simulink model "furuta_pi_motor_speed_a2"  (R2026b)
settings: Solver=FixedStepDiscrete  StopTime=inf  FixedStep=0.005  EnableMultiTasking=on
model workspace (MAT data in the model file):
  calibration = [nan -1 4058.5 1]
  drive = [0 0 0 0]
  limits = [0 0 15 0]
  motorSpeedRPM = Simulink.Parameter
  motorSpeedRPM.Value = 0
  motorSpeedRPM.Complexity = 'real'
  motorSpeedRPM.Dimensions = [1 1]
  motorSpeedRPM.CoderInfo.StorageClass = 'ExportedGlobal'
  motorSpeedRPM.DataType = 'double'
  speedSettings = [0 inf]
libraries: raspberrypiCommlib x5
settings Model: Creator=Lsh  LastModifiedBy=Lsh
settings SolverCC: PositivePriorityOrder=on
settings OptimizationCC: DifferentSizesBufferReuse=on  EfficientTunableParamExpr=on  EnhancedBackFolding=on  MaxStackSize=200000  OptimizationCustomize=off  OptimizeBlockOrder=speed  PassReuseOutputArgsAs=Individual arguments  RemoveInternalMemoryZeroInit=on  RemoveRootLevelIOMemoryZeroInit=on
settings DebuggingCC: ParameterTunabilityLossMsg=error
settings HardwareCC: ProdHWDeviceType=ARM Compatible->ARM Cortex-A (64-bit)  ProdLargestAtomicFloat=Double  ProdLargestAtomicInteger=LongLong  ProdLongLongMode=on
settings RTWCC: BuildConfiguration=Faster Runs  Description=Embedded Coder  HardwareBoard=Raspberry Pi (64bit)  SystemTargetFile=ert.tlc  TLCOptions="-aInlineSetEventsForThisBaseRateFcn=TLC_FALSE -aSuppressMultiTaskScheduler=TLC_FALSE  -aRateBasedStepFcn=0"  TemplateMakefile=ert_default_tmf  Toolchain=GNU GCC RPIUtils
settings CodeAppCC: ForceParamTrailComments=on  IgnoreCustomStorageClasses=off  InsertBlockDesc=on  OperatorAnnotations=on  SFDataObjDesc=on  SimulinkDataObjDesc=on
settings ERTTargetCC: CombineSignalStateStructs=on  ExtModeIntrfLevel=Level2 - Open  ExtModeMexFile=ext_xcp  ExtModeStaticAlloc=on  SupportVariableSizeSignals=on

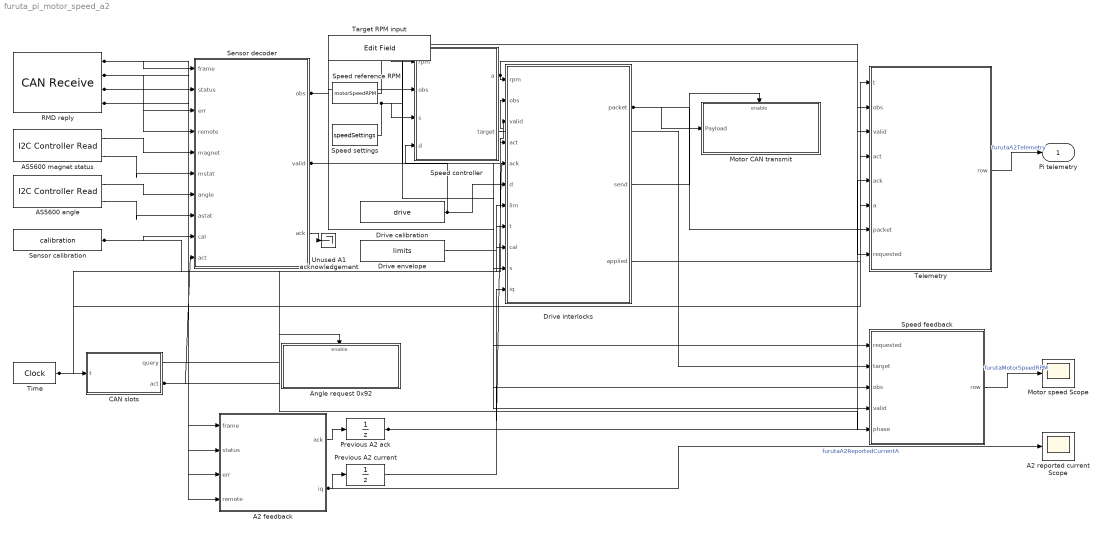
== system furuta_pi_motor_speed_a2 ==
  A2 feedback : MATLAB Function  TreatAsAtomicUnit=on
  A2 reported current Scope : Scope
  AS5600 angle : raspberrypiCommlib/I2C Controller Read  BoardProperty=Pi 5 Model  I2CModule=1  Mode=Master  SlaveAddress=54  SlaveByteOrder=BigEndian  Direction=Receiver  RegisterAddressMode=on  RegisterAddress=14  SlaveDataType=uint8  DataLength=2  NoAck=off  RepeatedStart=on  OutputStatus=on  SampleTime=.005
  AS5600 magnet status : raspberrypiCommlib/I2C Controller Read  BoardProperty=Pi 5 Model  I2CModule=1  Mode=Master  SlaveAddress=54  SlaveByteOrder=BigEndian  Direction=Receiver  RegisterAddressMode=on  RegisterAddress=11  SlaveDataType=uint8  DataLength=1  NoAck=off  RepeatedStart=on  OutputStatus=on  SampleTime=.005
  Angle request 0x92 : Subsystem  TreatAsAtomicUnit=on
  CAN slots : MATLAB Function  TreatAsAtomicUnit=on
  Drive calibration : Constant  Value=drive  SampleTime=.005
  Drive envelope : Constant  Value=limits  SampleTime=.005
  Drive interlocks : MATLAB Function  TreatAsAtomicUnit=on
  Motor CAN transmit : Subsystem  TreatAsAtomicUnit=on
  Motor speed Scope : Scope
  Previous A2 ack : UnitDelay  InitialCondition=false  SampleTime=.005
  Previous A2 current : UnitDelay  InitialCondition=NaN  SampleTime=.005
  RMD reply : raspberrypiCommlib/CAN Receive  DeviceID=can0  SetupCAN=off  TypeofCAN=Real  OutputDataType=Raw data  IdentifierType=Standard (11-bit identifier)  MessageId=577  MsgLength=8  SampleTime=.005  OutputError=on  OutputRemote=on  SimulateUsing=Code generation
  Sensor calibration : Constant  Value=calibration  SampleTime=.005
  Sensor decoder : MATLAB Function  TreatAsAtomicUnit=on
  Speed controller : MATLAB Function  TreatAsAtomicUnit=on
  Speed feedback : MATLAB Function  TreatAsAtomicUnit=on
  Speed reference RPM : Constant  Value=motorSpeedRPM  SampleTime=.005
  Speed settings : Constant  Value=speedSettings  SampleTime=.005
  Target RPM input : EditField  LabelPosition=Hide  ShowInitialText=on  Alignment=Center
  Telemetry : MATLAB Function  TreatAsAtomicUnit=on
  Time : DigitalClock  SampleTime=.005
  Unused A1 acknowledgement : Terminator
  Pi telemetry : Outport
  wires:
  Time/1 -> CAN slots/1(t), Drive interlocks/8(t), Telemetry/1(t)
  CAN slots/1(query) -> Angle request 0x92/Enable
  RMD reply/1 -> A2 feedback/1(frame), Sensor decoder/1(frame)
  RMD reply/2 -> A2 feedback/2(status), Sensor decoder/2(status)
  RMD reply/3 -> A2 feedback/3(err), Sensor decoder/3(err)
  RMD reply/4 -> A2 feedback/4(remote), Sensor decoder/4(remote)
  A2 feedback/1(ack) -> Previous A2 ack/1
  A2 feedback/2(iq) -> Previous A2 current/1, A2 reported current Scope/1  "furutaA2ReportedCurrentA"
  Sensor decoder/3(ack) -> Unused A1 acknowledgement/1
  AS5600 magnet status/1 -> Sensor decoder/5(magnet)
  AS5600 magnet status/2 -> Sensor decoder/6(mstat)
  AS5600 angle/1 -> Sensor decoder/7(angle)
  AS5600 angle/2 -> Sensor decoder/8(astat)
  Sensor calibration/1 -> Sensor decoder/9(cal), Drive interlocks/9(cal)
  CAN slots/2(act) -> Sensor decoder/10(act), Drive interlocks/4(act), Speed feedback/5(phase), Telemetry/4(act)
  Speed reference RPM/1 -> Speed controller/1(rpm), Speed feedback/1(requested)
  Sensor decoder/1(obs) -> Speed controller/2(obs), Drive interlocks/2(obs), Speed feedback/3(obs), Telemetry/2(obs)
  Speed settings/1 -> Speed controller/3(s), Drive interlocks/10(s)
  Drive calibration/1 -> Speed controller/4(d), Drive interlocks/6(d)
  Speed controller/1(a) -> Drive interlocks/1(rpm), Telemetry/8(requested)
  Sensor decoder/2(valid) -> Drive interlocks/3(valid), Speed feedback/4(valid), Telemetry/3(valid)
  Previous A2 ack/1 -> Drive interlocks/5(ack), Telemetry/5(ack)
  Drive envelope/1 -> Drive interlocks/7(lim)
  Previous A2 current/1 -> Drive interlocks/11(iq)
  Drive interlocks/1(packet) -> Motor CAN transmit/1(Payload), Telemetry/7(packet)
  Drive interlocks/2(send) -> Motor CAN transmit/Enable
  Speed controller/2(target) -> Speed feedback/2(target)
  Speed feedback/1(row) -> Motor speed Scope/1  "furutaMotorSpeedRPM"
  Drive interlocks/3(applied) -> Telemetry/6(a)
  Telemetry/1(row) -> Pi telemetry/1  "furutaA2Telemetry"

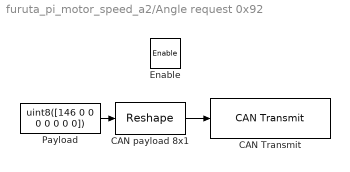
== system furuta_pi_motor_speed_a2/Angle request 0x92 ==
  Enable : EnablePort
  CAN Transmit : raspberrypiCommlib/CAN Transmit  DeviceID=can0  SetupCAN=off  TypeofCAN=Real  InputDataType=Raw data  BlockingMode_=off  BlockTimeout_=1  OutputStatus=off  IdentifierType=Standard (11-bit identifier)  MessageId=321  MsgLength=8  RemoteFrame=off  SimulateUsing=Code generation
  CAN payload 8x1 : Reshape  OutputDimensionality=Customize  OutputDimensions=[8 1]
  Payload : Constant  Value=uint8([146 0 0 0 0 0 0 0])  SampleTime=.005
  wires:
  Payload/1 -> CAN payload 8x1/1
  CAN payload 8x1/1 -> CAN Transmit/1

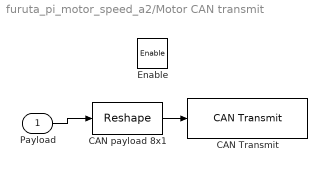
== system furuta_pi_motor_speed_a2/Motor CAN transmit ==
  Payload : Inport
  Enable : EnablePort
  CAN Transmit : raspberrypiCommlib/CAN Transmit  DeviceID=can0  SetupCAN=off  TypeofCAN=Real  InputDataType=Raw data  BlockingMode_=off  BlockTimeout_=1  OutputStatus=off  IdentifierType=Standard (11-bit identifier)  MessageId=321  MsgLength=8  RemoteFrame=off  SimulateUsing=Code generation
  CAN payload 8x1 : Reshape  OutputDimensionality=Customize  OutputDimensions=[8 1]
  wires:
  Payload/1 -> CAN payload 8x1/1
  CAN payload 8x1/1 -> CAN Transmit/1

== matlab function furuta_pi_motor_speed_a2/Sensor decoder ==
  data: frame input; obs output; status input; err input; remote input; magnet input; mstat input; angle input; astat input; cal input; act input; valid output; ack output
function [obs,valid,ack] = decode(frame,status,err,remote,magnet,mstat,angle,astat,cal,act)
[obs,valid,ack] = furuta_pi_sample(frame,status,err,remote,magnet,mstat,angle,astat,cal,act);
end

== matlab function furuta_pi_motor_speed_a2/CAN slots ==
  data: t input; query output; act output
function [query,act] = slots(t)
act = mod(round(t/.005),2)==1;
query = ~act;
end

== matlab function furuta_pi_motor_speed_a2/A2 feedback ==
  data: frame input; ack output; status input; err input; remote input; iq output
function [ack,iq] = feedback(frame,status,err,remote)
ack=frame(1)==162 && status==1 && err==0 && remote==0;
iq=NaN;
if ack
    counts=double(frame(3))+256*double(frame(4));
    if counts>=32768, counts=counts-65536; end
    iq=counts/100;
end
end

== matlab function furuta_pi_motor_speed_a2/Speed controller ==
  data: rpm input; a output; obs input; s input; d input; target output
function [a,target] = control(rpm,obs,s,d)
a = 0;
target = max(-s(2),min(s(2),rpm));
if ~isfinite(rpm), a = NaN; target = NaN; return, end
a = target;
end

== matlab function furuta_pi_motor_speed_a2/Drive interlocks ==
  data: rpm input; packet output; obs input; valid input; act input; ack input; d input; lim input; t input; cal input; s input; iq input; send output; applied output
function [packet,send,applied] = command(rpm,obs,valid,act,ack,d,lim,t,cal,s,iq)
persistent needsAck
if isempty(needsAck), needsAck = false; end
packet = zeros(1,8,'uint8'); send = false; applied = 0;
if ~act || d(4)==0, return, end
ok = valid && (~needsAck || (ack && isfinite(iq) && abs(iq)<=d(3)));
armed = valid || needsAck || t>.2;
[packet,send,applied] = furuta_pi_speed_frame(rpm,obs,ok,armed,cal(2),s(2),s(1),lim,t,d(4));
needsAck = packet(1)==162;
end

== matlab function furuta_pi_motor_speed_a2/Speed feedback ==
  data: requested input; row output; target input; obs input; valid input; phase input
function row = feedback(requested,target,obs,valid,phase)
persistent measured
if isempty(measured), measured = NaN; end
if phase
    measured = NaN;
    if valid, measured = obs(4)*60/(2*pi); end
end
row = [requested;target;measured];
end

== matlab function furuta_pi_motor_speed_a2/Telemetry ==
  data: t input; row output; obs input; valid input; act input; ack input; a input; packet input; requested input
function row = logrow(t,obs,valid,act,ack,a,packet,requested)
row = [t; double(act); double(valid); obs; a; double(packet(1)); double(ack); double(requested)];
end
